simulink model "MCS"  (R2018a)
settings: Solver=VariableStepAuto  StartTime=0.0  StopTime=0.2  RelTol=1e-3
libraries: powerlib x27, powerlib_meascontrol x1
settings Model: Creator=Acer  LastModifiedBy=Acer
settings DataIOCC: ReturnWorkspaceOutputs=on
settings DebuggingCC: UnconnectedInputMsg=none  UnconnectedOutputMsg=none  UnconnectedLineMsg=none
settings ModelReferenceCC: EnableRefExpFcnMdlSchedulingChecks=off
settings SFSimCC: SimUseLocalCustomCode=on
settings RTWCC: Description=Generic Real-Time Target  RTWUseLocalCustomCode=on

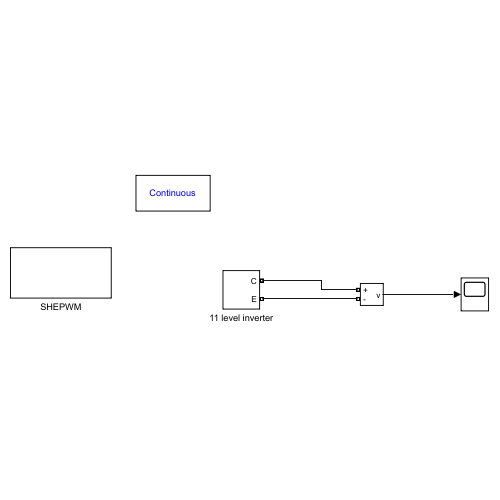
[thumbnail: Simulink's stored preview of the top-level diagram]
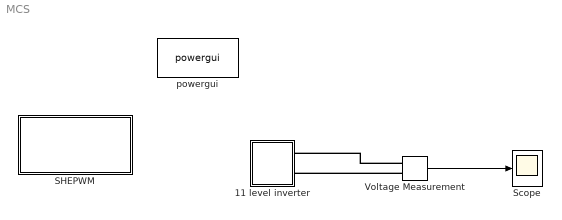
== system MCS ==
  11 level inverter : Subsystem
  SHEPWM : Subsystem
  Scope : Scope
  Voltage Measurement : powerlib/Measurements/Voltage Measurement  PhasorSimulation=off  OutputType=Complex  PSBequivalent=0
  powergui : powerlib/powergui  Priority=1  SimulationMode=Continuous  SampleTime=50e-6  frequency=60  Iterations=50  frequencyindice=0  Pbase=100e6  ErrMax=1e-4  UnitsV=kV  UnitsW=MW  buscounter=0  FunctionMessages=off  echomessages=off  EnableUseOfTLC=off  CurrentSourceSwitches=off  DisableSnubberDevices=off  DisableRonSwitches=off  DisableVfSwitches=off  DisplayEquations=off  AutomaticDiscreteSolvers=off  SolverType=Tustin/Backward Euler (TBE)  Interpol=off  ExternalGateDelay=off  methode=off  Ts=100  x0status=blocks  SPID=on  SwTol=0  HookPort=off  NonlinearTolerance=1e-4  nMaxIteration=100  ContinueOnMaxIteration=off  RestoreLinks=warning  ResistiveCurrentMeasurement=off  Frange=[0:2:500]  Ylog=off  Xlog=on  ShowGrid=off  save=off  variable=ZData  structure=0  ZoomFFT=off  StartTime=0.0  cycles=1  DisplayStyle=1  fundamental=60  FreqAxis=off  MaxFrequency=1000  frequencyindicesteady=1  RmsSteady=1  display=off
  wires:
  Voltage Measurement/1 -> Scope/1
  connections:
  Voltage Measurement/LConn2 -- 11 level inverter/RConn2
  Voltage Measurement/LConn1 -- 11 level inverter/RConn1

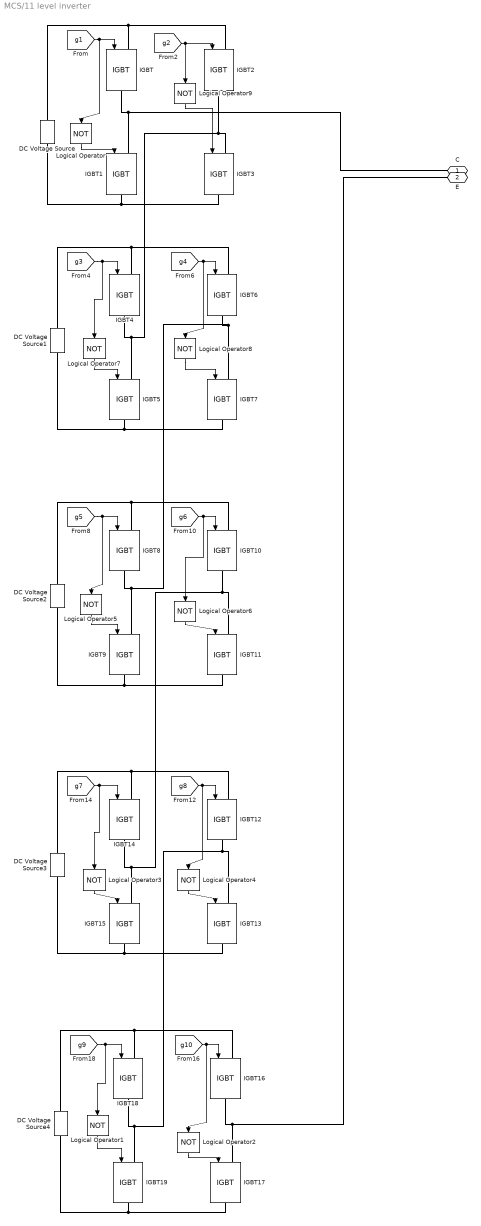
== system MCS/11 level inverter ==
  DC Voltage Source{,1..4} (5 alike) : powerlib/Electrical Sources/DC Voltage Source  Amplitude=100  Measurements=None
  IGBT{,1..19} (20 alike) : powerlib/Power Electronics/IGBT  Ron=0.001  Lon=0  Vf=1  Tf=1e-6  Tt=2e-6  IC=0  Rs=1e5  Cs=inf  Measurements=off
  Logical Operator{,1..9} (10 alike) : Logic  Operator=NOT  AllPortsSameDT=off  OutDataTypeStr=boolean
  C : PMIOPort  Side=Right
  E : PMIOPort  Port=2  Side=Right
  wires:
  [g8] -> Logical Operator4/1, IGBT12/1
  [g7] -> Logical Operator3/1, IGBT14/1
  Logical Operator9/1 -> IGBT3/1
  [g10] -> IGBT16/1, Logical Operator2/1
  [g5] -> IGBT8/1, Logical Operator5/1
  [g4] -> Logical Operator8/1, IGBT6/1
  Logical Operator1/1 -> IGBT19/1
  [g2] -> IGBT2/1, Logical Operator9/1
  Logical Operator4/1 -> IGBT13/1
  [g1] -> Logical Operator/1, IGBT/1
  [g3] -> IGBT4/1, Logical Operator7/1
  [g9] -> IGBT18/1, Logical Operator1/1
  Logical Operator/1 -> IGBT1/1
  [g6] -> IGBT10/1, Logical Operator6/1
  Logical Operator8/1 -> IGBT7/1
  Logical Operator7/1 -> IGBT5/1
  Logical Operator5/1 -> IGBT9/1
  Logical Operator3/1 -> IGBT15/1
  Logical Operator6/1 -> IGBT11/1
  Logical Operator2/1 -> IGBT17/1
  connections:
  IGBT10/RConn1 -- IGBT11/LConn1 -- IGBT14/RConn1 -- IGBT15/LConn1
  DC Voltage Source1/LConn1 -- IGBT7/RConn1 -- IGBT5/RConn1
  IGBT19/LConn1 -- IGBT13/LConn1 -- IGBT12/RConn1 -- IGBT18/RConn1
  IGBT6/LConn1 -- DC Voltage Source1/RConn1 -- IGBT4/LConn1
  IGBT5/LConn1 -- IGBT4/RConn1 -- IGBT3/LConn1 -- IGBT2/RConn1
  IGBT12/LConn1 -- DC Voltage Source3/RConn1 -- IGBT14/LConn1
  IGBT6/RConn1 -- IGBT8/RConn1 -- IGBT9/LConn1 -- IGBT7/LConn1
  IGBT2/LConn1 -- DC Voltage Source/RConn1 -- IGBT/LConn1
  IGBT10/LConn1 -- DC Voltage Source2/RConn1 -- IGBT8/LConn1
  DC Voltage Source4/LConn1 -- IGBT17/RConn1 -- IGBT19/RConn1
  DC Voltage Source2/LConn1 -- IGBT11/RConn1 -- IGBT9/RConn1
  IGBT/RConn1 -- C/RConn1 -- IGBT1/LConn1
  IGBT18/LConn1 -- DC Voltage Source4/RConn1 -- IGBT16/LConn1
  IGBT17/LConn1 -- E/RConn1 -- IGBT16/RConn1
  DC Voltage Source/LConn1 -- IGBT3/RConn1 -- IGBT1/RConn1
  DC Voltage Source3/LConn1 -- IGBT13/RConn1 -- IGBT15/RConn1

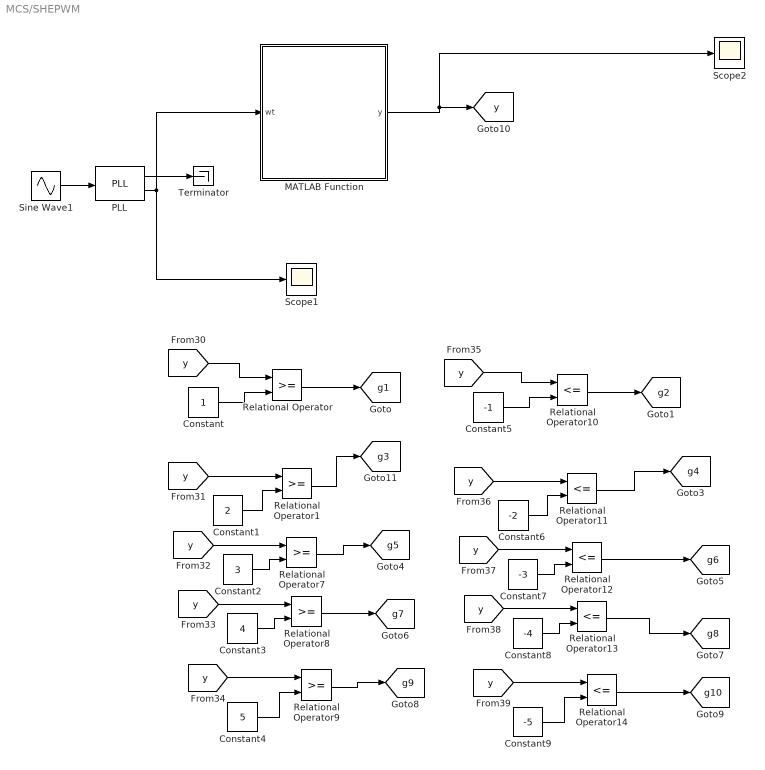
== system MCS/SHEPWM ==
  Constant : Constant
  Constant1 : Constant  Value=2
  Constant2 : Constant  Value=3
  Constant3 : Constant  Value=4
  Constant4 : Constant  Value=5
  Constant5 : Constant  Value=-1
  Constant6 : Constant  Value=-2
  Constant7 : Constant  Value=-3
  Constant8 : Constant  Value=-4
  Constant9 : Constant  Value=-5
  MATLAB Function : MATLAB Function  TreatAsAtomicUnit=on
  PLL : powerlib_meascontrol/PLL/PLL  Fmin=45  Par_Init=[0, 50]  ParK=[180, 3200, 1]  TcD=1e-4  MaxRateChangeFreq=12  FilterCutOffFreq=25  Ts=0  AGC=on
  Relational Operator{,1,7..9} (5 alike) : RelationalOperator  OutDataTypeStr=boolean  RndMeth=Simplest
  Relational Operator{10..14} (5 alike) : RelationalOperator  Operator=<=  OutDataTypeStr=boolean  RndMeth=Simplest
  Scope1 : Scope
  Scope2 : Scope
  Sine Wave1 : Sin  Frequency=2*pi*50  SampleTime=0
  Terminator : Terminator
  tag scope: g10=global, g1=global, g2=global, g3=global, g4=global, g5=global, g6=global, g7=global, g8=global, g9=global, y=global
  wires:
  Relational Operator14/1 -> [g10]
  [y] -> Relational Operator11/1
  Constant1/1 -> Relational Operator1/2
  Relational Operator/1 -> [g1]
  [y] -> Relational Operator14/1
  PLL/2 -> Scope1/1, MATLAB Function/1(wt)
  MATLAB Function/1(y) -> Scope2/1, [y]
  Relational Operator12/1 -> [g6]
  Constant7/1 -> Relational Operator12/2
  [y] -> Relational Operator10/1
  Sine Wave1/1 -> PLL/1
  Constant9/1 -> Relational Operator14/2
  Relational Operator13/1 -> [g8]
  Relational Operator7/1 -> [g5]
  [y] -> Relational Operator7/1
  Relational Operator8/1 -> [g7]
  [y] -> Relational Operator9/1
  [y] -> Relational Operator1/1
  Constant8/1 -> Relational Operator13/2
  Relational Operator10/1 -> [g2]
  Relational Operator11/1 -> [g4]
  [y] -> Relational Operator12/1
  Relational Operator9/1 -> [g9]
  Constant5/1 -> Relational Operator10/2
  Constant/1 -> Relational Operator/2
  PLL/1 -> Terminator/1
  Constant4/1 -> Relational Operator9/2
  Constant6/1 -> Relational Operator11/2
  Constant2/1 -> Relational Operator7/2
  Constant3/1 -> Relational Operator8/2
  [y] -> Relational Operator13/1
  [y] -> Relational Operator8/1
  Relational Operator1/1 -> [g3]
  [y] -> Relational Operator/1

== matlab function MCS/SHEPWM/MATLAB Function ==
  data: wt input; y output
function y = she_pwm_11level_7th(wt)
    % Optimal switching angles for 11-level, 7th harmonic elimination (degrees)
    % These angles are precomputed for M = 0.8
    angles_deg =[6.57, 18.94, 27.18, 45.15, 62.24];
    alpha = (angles_deg * pi/180); % Convert to radians and sort
    
    % Normalize angle to [0, 2π)
    %wt = mod(wt, 2*pi);
    y = 0;
    
    % Positive half-cycle (0 to π)
    if wt < pi
        % Determine which bridges should be active
        if wt >= alpha(5) && wt < pi - alpha(5)
            y = 5; % All 5 bridges positive
        elseif wt >= alpha(4) && wt < pi - alpha(4)
            y = 4; % 4 bridges positive
        elseif wt >= alpha(3) && wt < pi - alpha(3)
            y = 3; % 3 bridges positive
        elseif wt >= alpha(2) && wt < pi - alpha(2)
            y = 2; % 2 bridges positive
        elseif wt >= alpha(1) && wt < pi - alpha(1)
            y = 1; % 1 bridge positive
        end
    % Negative half-cycle (π to 2π)
    else
        % Determine which bridges should be active
        if wt >= pi + alpha(5) && wt < 2*pi - alpha(5)
            y = -5; % All 5 bridges negative
        elseif wt >= pi + alpha(4) && wt < 2*pi - alpha(4)
            y = -4; % 4 bridges negative
        elseif wt >= pi + alpha(3) && wt < 2*pi - alpha(3)
            y = -3; % 3 bridges negative
        elseif wt >= pi + alpha(2) && wt < 2*pi - alpha(2)
            y = -2; % 2 bridges negative
        elseif wt >= pi + alpha(1) && wt < 2*pi - alpha(1)
            y = -1; % 1 bridge negative
        end
    end
end
